simulink model "Architecture_261027_ver9"  (R2026b)
settings: Solver=FixedStepDiscrete  FixedStep=0.005
(part 1 of 2)
settings Model: DataDictionary=Architecture_ver00_dict.sldd  Creator=user  LastModifiedBy=user
settings OptimizationCC: DefaultParameterBehavior=Inlined  DifferentSizesBufferReuse=on  EfficientFloat2IntCast=on  EfficientTunableParamExpr=on  GainParamInheritBuiltInType=on  InlineInvariantSignals=on  LifeSpan=1  NoFixptDivByZeroProtection=on  OptimizeBlockOrder=speed  PassReuseOutputArgsAs=Individual arguments  RemoveInternalMemoryZeroInit=on  RemoveRootLevelIOMemoryZeroInit=on  UseDivisionForNetSlopeComputation=on  UseFloatMulNetSlope=on
settings DebuggingCC: ParameterTunabilityLossMsg=error
settings HardwareCC: ProdHWDeviceType=Infineon->TriCore  ProdLargestAtomicFloat=None  ProdLongLongMode=on
settings SFSimCC: MATLABDynamicMemAlloc=off
settings RTWCC: DataTypeReplacement=CDataTypesFixedWidth  Description=Embedded Coder  GPUComputeCapability=5.0  GenCodeOnly=on  SystemTargetFile=ert.tlc  TemplateMakefile=ert_default_tmf
settings CodeAppCC: ForceParamTrailComments=on  IgnoreCustomStorageClasses=off  InsertBlockDesc=on  OperatorAnnotations=on  SFDataObjDesc=on  SimulinkDataObjDesc=on
settings ERTTargetCC: CombineSignalStateStructs=on  ERTFilePackagingFormat=CompactWithDataFile  IncludeMdlTerminateFcn=off  MaxIdInt16=INT16_MAX  MaxIdInt32=INT32_MAX  MaxIdInt64=INT64_MAX  MaxIdInt8=INT8_MAX  MaxIdUint16=UINT16_MAX  MaxIdUint32=UINT32_MAX  MaxIdUint64=UINT64_MAX  MaxIdUint8=UINT8_MAX  MinIdInt16=INT16_MIN  MinIdInt32=INT32_MIN  MinIdInt64=INT64_MIN  MinIdInt8=INT8_MIN  SupportAbsoluteTime=off  SupportComplex=off  SupportNonFinite=off  SuppressErrorStatus=on

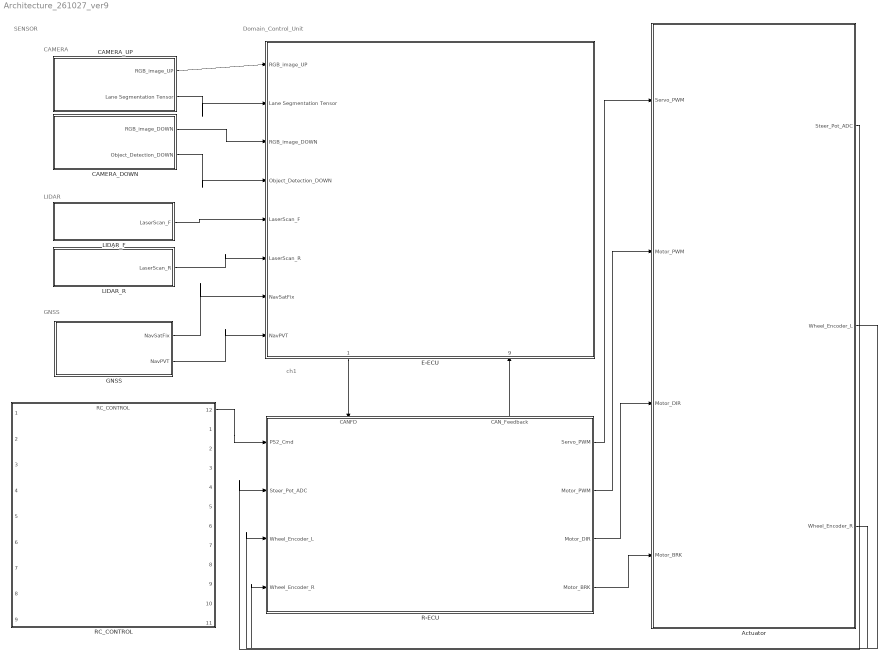
== system Architecture_261027_ver9 ==
  note: ch1
  note: Domain_Control_Unit
  note: SENSOR
  note: CAMERA
  note: GNSS
  note: LIDAR
  Actuator : Subsystem
      settings: PortSchema="{\"entries\":[{\"content\":{\"headerSize\":26,\"margin\":15,\"minimumSpacing\":25,\"sides\":[{\"content\":{\"connectorIds\":[\"In1\",\"In2\",\"In4\",\"In3\"]},\"type\":\"ConnectorPlacement.EquallySpacedRectSide\",\"uuid\":\"5be6b78a-1fb5-4892-a059-20486cb8da03\"},{\"content\":{\"connectorIds\":[\"Out2\",\"Out1\",\"Out3\"],\"side\":\"RIGHT\"},\"type\":\"ConnectorPlacement.EquallySpacedRectSide\",\"uuid\":\"6033bdc5-529e-4fd7-96df-de1a61a0c34f\"},{\"content\":{\"side\":\"TOP\"},\"type\":\"ConnectorPlacement.EquallySpacedRectSide\",\"uuid\":\"4d265f78-1951-4f58-a661-9dd8a9ad83fa\"}]},\"type\":\"ConnectorPlacement.EquallySpacedConnector\",\"uuid\":\"a5be31a5-398c-4cfa-a3f1-90989462f386\"}],\"packageUris\":[\"http://schema.mathworks.com/mf0/Connector/R2020b\"],\"version\":\"1.0\"}"
  CAMERA_DOWN : Subsystem
      settings: PortSchema="{\"entries\":[{\"content\":{\"headerSize\":26,\"margin\":15,\"minimumSpacing\":25,\"sides\":[{\"content\":{},\"type\":\"ConnectorPlacement.EquallySpacedRectSide\",\"uuid\":\"5be6b78a-1fb5-4892-a059-20486cb8da03\"},{\"content\":{\"connectorIds\":[\"Out1\",\"Out2\"],\"side\":\"RIGHT\"},\"type\":\"ConnectorPlacement.EquallySpacedRectSide\",\"uuid\":\"6033bdc5-529e-4fd7-96df-de1a61a0c34f\"},{\"content\":{\"side\":\"TOP\"},\"type\":\"ConnectorPlacement.EquallySpacedRectSide\",\"uuid\":\"4d265f78-1951-4f58-a661-9dd8a9ad83fa\"}]},\"type\":\"ConnectorPlacement.EquallySpacedConnector\",\"uuid\":\"a5be31a5-398c-4cfa-a3f1-90989462f386\"}],\"packageUris\":[\"http://schema.mathworks.com/mf0/Connector/R2020b\"],\"version\":\"1.0\"}"
  CAMERA_UP : Subsystem
      settings: PortSchema="{\"entries\":[{\"content\":{\"headerSize\":26,\"margin\":15,\"minimumSpacing\":25,\"sides\":[{\"content\":{},\"type\":\"ConnectorPlacement.EquallySpacedRectSide\",\"uuid\":\"5be6b78a-1fb5-4892-a059-20486cb8da03\"},{\"content\":{\"connectorIds\":[\"Out1\",\"Out2\"],\"side\":\"RIGHT\"},\"type\":\"ConnectorPlacement.EquallySpacedRectSide\",\"uuid\":\"6033bdc5-529e-4fd7-96df-de1a61a0c34f\"},{\"content\":{\"side\":\"TOP\"},\"type\":\"ConnectorPlacement.EquallySpacedRectSide\",\"uuid\":\"4d265f78-1951-4f58-a661-9dd8a9ad83fa\"}]},\"type\":\"ConnectorPlacement.EquallySpacedConnector\",\"uuid\":\"a5be31a5-398c-4cfa-a3f1-90989462f386\"}],\"packageUris\":[\"http://schema.mathworks.com/mf0/Connector/R2020b\"],\"version\":\"1.0\"}"
  E-ECU : Subsystem
      settings: PortSchema="{\"entries\":[{\"content\":{\"headerSize\":26,\"margin\":15,\"minimumSpacing\":25,\"sides\":[{\"content\":{\"connectorIds\":[\"In1\",\"In2\",\"In3\",\"In4\",\"In5\",\"In6\",\"In7\",\"In8\"]},\"type\":\"ConnectorPlacement.EquallySpacedRectSide\",\"uuid\":\"10eeddd2-005b-4c36-905d-85150b5a76ba\"},{\"content\":{\"side\":\"RIGHT\"},\"type\":\"ConnectorPlacement.EquallySpacedRectSide\",\"uuid\":\"bedc3a09-ff49-49cc-a7fa-ee3f02f55a8a\"},{\"content\":{\"side\":\"TOP\"},\"type\":\"ConnectorPlacement.EquallySpacedRectSide\",\"uuid\":\"08175ed9-a39d-44a1-a51d-de8180bc2cb7\"},{\"content\":{\"connectorIds\":[\"Out1\",\"In9\"],\"side\":\"BOTTOM\"},\"type\":\"ConnectorPlacement.EquallySpacedRectSide\",\"uuid\":\"733d255f-bca5-45f8-986d-3d6c4c00fa39\"}]},\"type\":\"ConnectorPlacement.EquallySpacedConnector\",\"uuid\":\"c3651b75-d651-4d18-be21-a5b7754dce1a\"}],\"packageUris\":[\"http://schema.mathworks.com/mf0/Connector/R2020b\"],\"version\":\"1.0\"}"
  GNSS : Subsystem
      settings: PortSchema="{\"entries\":[{\"content\":{\"headerSize\":26,\"margin\":15,\"minimumSpacing\":25,\"sides\":[{\"content\":{},\"type\":\"ConnectorPlacement.EquallySpacedRectSide\",\"uuid\":\"5be6b78a-1fb5-4892-a059-20486cb8da03\"},{\"content\":{\"connectorIds\":[\"Out1\",\"Out2\"],\"side\":\"RIGHT\"},\"type\":\"ConnectorPlacement.EquallySpacedRectSide\",\"uuid\":\"6033bdc5-529e-4fd7-96df-de1a61a0c34f\"},{\"content\":{\"side\":\"TOP\"},\"type\":\"ConnectorPlacement.EquallySpacedRectSide\",\"uuid\":\"4d265f78-1951-4f58-a661-9dd8a9ad83fa\"}]},\"type\":\"ConnectorPlacement.EquallySpacedConnector\",\"uuid\":\"a5be31a5-398c-4cfa-a3f1-90989462f386\"}],\"packageUris\":[\"http://schema.mathworks.com/mf0/Connector/R2020b\"],\"version\":\"1.0\"}"
  LIDAR_F : Subsystem
      settings: PortSchema="{\"entries\":[{\"content\":{\"headerSize\":26,\"margin\":15,\"minimumSpacing\":25,\"sides\":[{\"content\":{},\"type\":\"ConnectorPlacement.EquallySpacedRectSide\",\"uuid\":\"5be6b78a-1fb5-4892-a059-20486cb8da03\"},{\"content\":{\"connectorIds\":[\"Out1\"],\"side\":\"RIGHT\"},\"type\":\"ConnectorPlacement.EquallySpacedRectSide\",\"uuid\":\"6033bdc5-529e-4fd7-96df-de1a61a0c34f\"},{\"content\":{\"side\":\"TOP\"},\"type\":\"ConnectorPlacement.EquallySpacedRectSide\",\"uuid\":\"4d265f78-1951-4f58-a661-9dd8a9ad83fa\"}]},\"type\":\"ConnectorPlacement.EquallySpacedConnector\",\"uuid\":\"a5be31a5-398c-4cfa-a3f1-90989462f386\"}],\"packageUris\":[\"http://schema.mathworks.com/mf0/Connector/R2020b\"],\"version\":\"1.0\"}"
  LIDAR_R : Subsystem
      settings: PortSchema="{\"entries\":[{\"content\":{\"headerSize\":26,\"margin\":15,\"minimumSpacing\":25,\"sides\":[{\"content\":{},\"type\":\"ConnectorPlacement.EquallySpacedRectSide\",\"uuid\":\"5be6b78a-1fb5-4892-a059-20486cb8da03\"},{\"content\":{\"connectorIds\":[\"Out1\"],\"side\":\"RIGHT\"},\"type\":\"ConnectorPlacement.EquallySpacedRectSide\",\"uuid\":\"6033bdc5-529e-4fd7-96df-de1a61a0c34f\"},{\"content\":{\"side\":\"TOP\"},\"type\":\"ConnectorPlacement.EquallySpacedRectSide\",\"uuid\":\"4d265f78-1951-4f58-a661-9dd8a9ad83fa\"}]},\"type\":\"ConnectorPlacement.EquallySpacedConnector\",\"uuid\":\"a5be31a5-398c-4cfa-a3f1-90989462f386\"}],\"packageUris\":[\"http://schema.mathworks.com/mf0/Connector/R2020b\"],\"version\":\"1.0\"}"
  R-ECU : Subsystem
      settings: PortSchema="{\"entries\":[{\"content\":{\"headerSize\":26,\"margin\":15,\"minimumSpacing\":25,\"sides\":[{\"content\":{\"connectorIds\":[\"In1\",\"In3\",\"In2\",\"In4\"]},\"type\":\"ConnectorPlacement.EquallySpacedRectSide\",\"uuid\":\"5be6b78a-1fb5-4892-a059-20486cb8da03\"},{\"content\":{\"connectorIds\":[\"Out2\",\"Out4\",\"Out3\",\"Out5\"],\"side\":\"RIGHT\"},\"type\":\"ConnectorPlacement.EquallySpacedRectSide\",\"uuid\":\"6033bdc5-529e-4fd7-96df-de1a61a0c34f\"},{\"content\":{\"connectorIds\":[\"In5\",\"Out1\"],\"side\":\"TOP\"},\"type\":\"ConnectorPlacement.EquallySpacedRectSide\",\"uuid\":\"4d265f78-1951-4f58-a661-9dd8a9ad83fa\"}]},\"type\":\"ConnectorPlacement.EquallySpacedConnector\",\"uuid\":\"a5be31a5-398c-4cfa-a3f1-90989462f386\"}],\"packageUris\":[\"http://schema.mathworks.com/mf0/Connector/R2020b\"],\"version\":\"1.0\"}"
  RC_CONTROL : ModelReference  ModelNameDialog=RC_CONTROL  SimulationMode=Normal  ModelReferenceVersion=1.10
      settings: PortSchema="{\"entries\":[{\"content\":{\"headerSize\":38,\"margin\":15,\"minimumSpacing\":25,\"sides\":[{\"content\":{\"connectorIds\":[\"In1\",\"In2\",\"In3\",\"In4\",\"In5\",\"In6\",\"In7\",\"In8\",\"In9\"]},\"type\":\"ConnectorPlacement.EquallySpacedRectSide\",\"uuid\":\"f8644c43-7de7-4551-975f-61d7214ac11a\"},{\"content\":{\"connectorIds\":[\"Out12\",\"Out1\",\"Out2\",\"Out3\",\"Out4\",\"Out5\",\"Out6\",\"Out7\",\"Out8\",\"Out9\",\"Out10\",\"Out11\"],\"side\":\"RIGHT\"},\"type\":\"ConnectorPlacement.EquallySpacedRectSide\",\"uuid\":\"f00a2047-0f06-437d-84ca-9ac4a3f2c44a\"},{\"content\":{\"side\":\"TOP\"},\"type\":\"ConnectorPlacement.EquallySpacedRectSide\",\"uuid\":\"162e5f72-53e9-4ab8-ad74-bc845fd36bb8\"}]},\"type\":\"ConnectorPlacement.EquallySpacedConnector\",\"uuid\":\"4927cb8c-a923-4407-aae2-156d09df746b\"}],\"packageUris\":[\"http://schema.mathworks.com/mf0/Connector/R2020b\"],\"version\":\"1.0\"}"
  wires:
  R-ECU/2(Servo_PWM) -> Actuator/1(Servo_PWM)
  R-ECU/4(Motor_PWM) -> Actuator/2(Motor_PWM)
  R-ECU/5(Motor_BRK) -> Actuator/3(Motor_BRK)
  Actuator/1(Wheel_Encoder_L) -> R-ECU/2(Wheel_Encoder_L)
  Actuator/2(Steer_Pot_ADC) -> R-ECU/3(Steer_Pot_ADC)
  R-ECU/1(CAN_Feedback) -> E-ECU/9("  ")
  E-ECU/1("   ") -> R-ECU/5(CANFD)
  Actuator/3(Wheel_Encoder_R) -> R-ECU/4(Wheel_Encoder_R)
  R-ECU/3(Motor_DIR) -> Actuator/4(Motor_DIR)
  LIDAR_F/1(LaserScan_F) -> E-ECU/5(LaserScan_F)
  LIDAR_R/1(LaserScan_R) -> E-ECU/6(LaserScan_R)
  GNSS/1("NavSatFix ") -> E-ECU/7("NavSatFix ")
  GNSS/2(NavPVT) -> E-ECU/8(NavPVT)
  CAMERA_UP/1(RGB_image_UP) -> E-ECU/1(RGB_image_UP)
  CAMERA_DOWN/1(RGB_image_DOWN) -> E-ECU/3(RGB_image_DOWN)
  CAMERA_DOWN/2(Object_Detection_DOWN) -> E-ECU/4(Object_Detection_DOWN)
  CAMERA_UP/2(Lane Segmentation Tensor) -> E-ECU/2(Lane Segmentation Tensor)
  RC_CONTROL/12 -> R-ECU/1(PS2_Cmd)

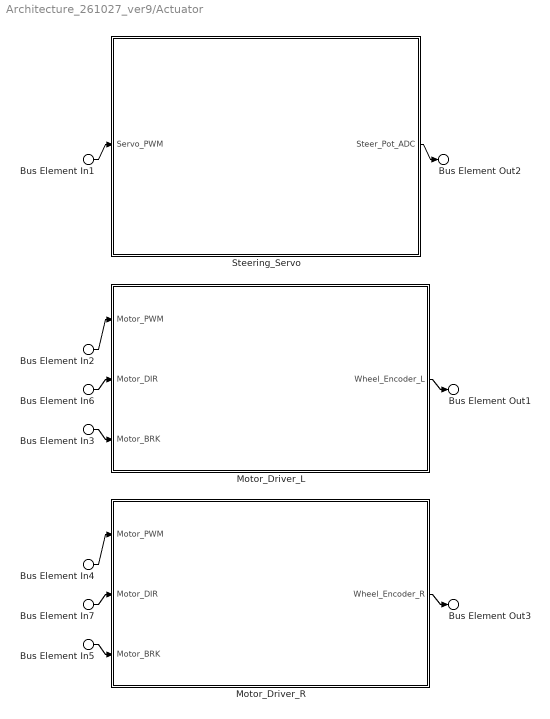
== system Architecture_261027_ver9/Actuator ==
  Bus Element In1 : Inport  PortName=Servo_PWM
  Bus Element In2 : Inport  Port=2  PortName=Motor_PWM
  Bus Element In4 : Inport  Port=2  PortName=Motor_PWM
  Bus Element In3 : Inport  Port=3  PortName=Motor_BRK
  Bus Element In5 : Inport  Port=3  PortName=Motor_BRK
  Bus Element In6 : Inport  Port=4  PortName=Motor_DIR
  Bus Element In7 : Inport  Port=4  PortName=Motor_DIR
  Motor_Driver_L : Subsystem
      settings: PortSchema="{\"entries\":[{\"content\":{\"headerSize\":26,\"margin\":15,\"minimumSpacing\":25,\"sides\":[{\"content\":{\"connectorIds\":[\"In1\",\"In2\",\"In3\"]},\"type\":\"ConnectorPlacement.EquallySpacedRectSide\",\"uuid\":\"5be6b78a-1fb5-4892-a059-20486cb8da03\"},{\"content\":{\"connectorIds\":[\"Out1\"],\"side\":\"RIGHT\"},\"type\":\"ConnectorPlacement.EquallySpacedRectSide\",\"uuid\":\"6033bdc5-529e-4fd7-96df-de1a61a0c34f\"},{\"content\":{\"side\":\"TOP\"},\"type\":\"ConnectorPlacement.EquallySpacedRectSide\",\"uuid\":\"4d265f78-1951-4f58-a661-9dd8a9ad83fa\"}]},\"type\":\"ConnectorPlacement.EquallySpacedConnector\",\"uuid\":\"a5be31a5-398c-4cfa-a3f1-90989462f386\"}],\"packageUris\":[\"http://schema.mathworks.com/mf0/Connector/R2020b\"],\"version\":\"1.0\"}"
  Motor_Driver_R : Subsystem
      settings: PortSchema="{\"entries\":[{\"content\":{\"headerSize\":26,\"margin\":15,\"minimumSpacing\":25,\"sides\":[{\"content\":{\"connectorIds\":[\"In1\",\"In2\",\"In3\"]},\"type\":\"ConnectorPlacement.EquallySpacedRectSide\",\"uuid\":\"5be6b78a-1fb5-4892-a059-20486cb8da03\"},{\"content\":{\"connectorIds\":[\"Out1\"],\"side\":\"RIGHT\"},\"type\":\"ConnectorPlacement.EquallySpacedRectSide\",\"uuid\":\"6033bdc5-529e-4fd7-96df-de1a61a0c34f\"},{\"content\":{\"side\":\"TOP\"},\"type\":\"ConnectorPlacement.EquallySpacedRectSide\",\"uuid\":\"4d265f78-1951-4f58-a661-9dd8a9ad83fa\"}]},\"type\":\"ConnectorPlacement.EquallySpacedConnector\",\"uuid\":\"a5be31a5-398c-4cfa-a3f1-90989462f386\"}],\"packageUris\":[\"http://schema.mathworks.com/mf0/Connector/R2020b\"],\"version\":\"1.0\"}"
  Steering_Servo : Subsystem
      settings: PortSchema="{\"entries\":[{\"content\":{\"headerSize\":26,\"margin\":15,\"minimumSpacing\":25,\"sides\":[{\"content\":{\"connectorIds\":[\"In1\"]},\"type\":\"ConnectorPlacement.EquallySpacedRectSide\",\"uuid\":\"5be6b78a-1fb5-4892-a059-20486cb8da03\"},{\"content\":{\"connectorIds\":[\"Out1\"],\"side\":\"RIGHT\"},\"type\":\"ConnectorPlacement.EquallySpacedRectSide\",\"uuid\":\"6033bdc5-529e-4fd7-96df-de1a61a0c34f\"},{\"content\":{\"side\":\"TOP\"},\"type\":\"ConnectorPlacement.EquallySpacedRectSide\",\"uuid\":\"4d265f78-1951-4f58-a661-9dd8a9ad83fa\"}]},\"type\":\"ConnectorPlacement.EquallySpacedConnector\",\"uuid\":\"a5be31a5-398c-4cfa-a3f1-90989462f386\"}],\"packageUris\":[\"http://schema.mathworks.com/mf0/Connector/R2020b\"],\"version\":\"1.0\"}"
  Bus Element Out1 : Outport  PortName=Wheel_Encoder_L
  Bus Element Out2 : Outport  Port=2  PortName=Steer_Pot_ADC
  Bus Element Out3 : Outport  Port=3  PortName=Wheel_Encoder_R
  wires:
  Motor_Driver_L/1(Wheel_Encoder_L) -> Bus Element Out1/1
  Bus Element In1/1 -> Steering_Servo/1(Servo_PWM)
  Bus Element In2/1 -> Motor_Driver_L/1(Motor_PWM)
  Bus Element In3/1 -> Motor_Driver_L/3(Motor_BRK)
  Steering_Servo/1(Steer_Pot_ADC) -> Bus Element Out2/1
  Motor_Driver_R/1(Wheel_Encoder_R) -> Bus Element Out3/1
  Bus Element In4/1 -> Motor_Driver_R/1(Motor_PWM)
  Bus Element In5/1 -> Motor_Driver_R/3(Motor_BRK)
  Bus Element In6/1 -> Motor_Driver_L/2(Motor_DIR)
  Bus Element In7/1 -> Motor_Driver_R/2(Motor_DIR)

== system Architecture_261027_ver9/CAMERA_DOWN ==
  Bus Element Out1 : Outport  PortName=RGB_image_DOWN
  Bus Element Out2 : Outport  Port=2  PortName=Object_Detection_DOWN

== system Architecture_261027_ver9/CAMERA_UP ==
  Bus Element Out1 : Outport  PortName=RGB_image_UP
  Bus Element Out2 : Outport  Port=2  PortName=Lane Segmentation Tensor

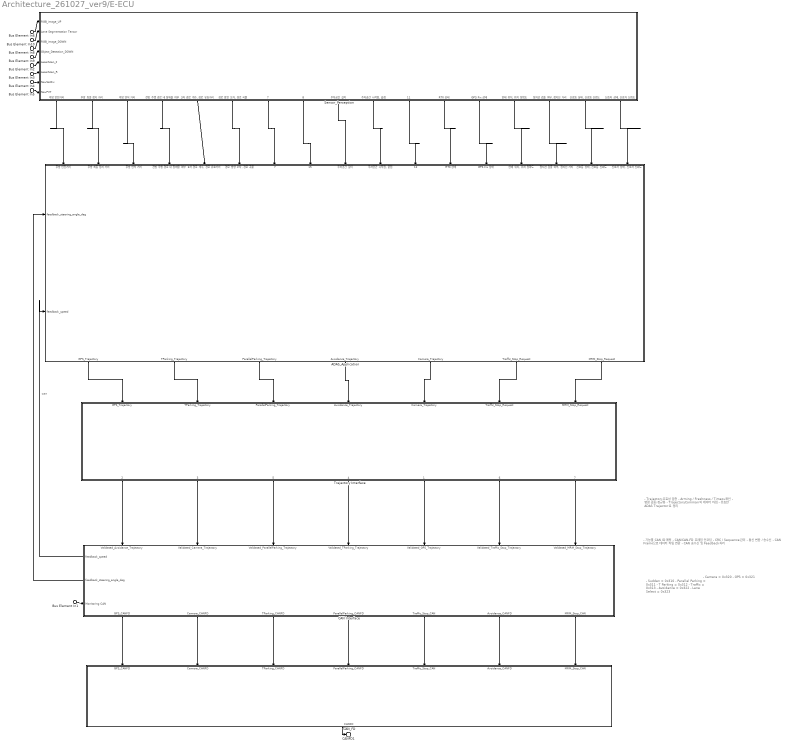
== system Architecture_261027_ver9/E-ECU ==
  note: can
  note: - 기능별 CAN ID 매핑
      | - CAN/CAN-FD 프레임 인코딩
      | - CRC / Sequence 관리
      | - 통신 변환 / 송수신
      | - CAN Frame으로 데이터 타입 변환
      | - CAN 송수신 및 Feedback 처리
  note: - Trajectory 유효성 검증
      | - Arming / Freshness / Timeout 확인
      | - 명령 검증/정규화
      | - TrajectoryCommand의 데이터 타입
      | - 유효한 ADAS Trajectory로 정리
  note: - Camera = 0x320
      | - GPS = 0x321
  note: - Sudden = 0x310
      | - Parallel Parking = 0x311
      | - T Parking = 0x312
      | - Traffic = 0x313
      | - Avoidance = 0x322
      | - Lane Select = 0x323
  Bus Element In6 : Inport  PortName=RGB_image_UP
  Bus Element In10 : Inport  Port=2  PortName=Lane Segmentation Tensor
  Bus Element In8 : Inport  Port=3  PortName=RGB_image_DOWN
  Bus Element In9 : Inport  Port=4  PortName=Object_Detection_DOWN
  Bus Element In2 : Inport  Port=5  PortName=LaserScan_F
  Bus Element In3 : Inport  Port=6  PortName=LaserScan_R
  Bus Element In4 : Inport  Port=7  PortName=NavSatFix
  Bus Element In5 : Inport  Port=8  PortName=NavPVT
  Bus Element In1 : Inport  Port=9  PortName=""
  ADAS_Application : Subsystem
      settings: PortSchema="{\"entries\":[{\"content\":{\"headerSize\":26,\"margin\":15,\"minimumSpacing\":25,\"sides\":[{\"content\":{\"connectorIds\":[\"In5\",\"In8\"]},\"type\":\"ConnectorPlacement.EquallySpacedRectSide\",\"uuid\":\"47be2e05-6379-4865-963e-e2af5bd447f4\"},{\"content\":{\"side\":\"RIGHT\"},\"type\":\"ConnectorPlacement.EquallySpacedRectSide\",\"uuid\":\"eee9a279-489d-42b1-868c-6501adb5baa4\"},{\"content\":{\"connectorIds\":[\"In19\",\"In18\",\"In17\",\"In16\",\"In4\",\"In6\",\"In7\",\"In15\",\"In14\",\"In13\",\"In12\",\"In11\",\"In10\",\"In9\",\"In2\",\"In1\",\"In3\"],\"side\":\"TOP\"},\"type\":\"ConnectorPlacement.EquallySpacedRectSide\",\"uuid\":\"1fb23197-7de0-4afe-988c-73e75d3e5644\"},{\"content\":{\"connectorIds\":[\"Out1\",\"Out2\",\"Out3\",\"Out4\",\"Out5\",\"Out7\",\"Out6\"],\"side\":\"BOTTOM\"},\"type\":\"ConnectorPlacement.EquallySpacedRectSide\",\"uuid\":\"4316405c-13a5-45fc-a271-26a0825c33e2\"}]},\"type\":\"ConnectorPlacement.EquallySpacedConnector\",\"uuid\":\"0ef4e16f-7381-4a8b-98d2-b00a0700ad12\"}],\"packageUris\":[\"http://schema.mathworks.com/mf0/Connector/R2020b\"],\"version\":\"1.0\"}"
  CAN Interface : Subsystem
      settings: PortSchema="{\"entries\":[{\"content\":{\"headerSize\":26,\"margin\":15,\"minimumSpacing\":25,\"sides\":[{\"content\":{\"connectorIds\":[\"Out1\",\"Out2\",\"In1\"]},\"type\":\"ConnectorPlacement.EquallySpacedRectSide\",\"uuid\":\"47be2e05-6379-4865-963e-e2af5bd447f4\"},{\"content\":{\"side\":\"RIGHT\"},\"type\":\"ConnectorPlacement.EquallySpacedRectSide\",\"uuid\":\"eee9a279-489d-42b1-868c-6501adb5baa4\"},{\"content\":{\"connectorIds\":[\"In8\",\"In3\",\"In5\",\"In4\",\"In2\",\"In6\",\"In7\"],\"side\":\"TOP\"},\"type\":\"ConnectorPlacement.EquallySpacedRectSide\",\"uuid\":\"1fb23197-7de0-4afe-988c-73e75d3e5644\"},{\"content\":{\"connectorIds\":[\"Out3\",\"Out4\",\"Out5\",\"Out6\",\"Out8\",\"Out7\",\"Out9\"],\"side\":\"BOTTOM\"},\"type\":\"ConnectorPlacement.EquallySpacedRectSide\",\"uuid\":\"b394a130-1425-4269-a0f2-9cc8deadb9ec\"}]},\"type\":\"ConnectorPlacement.EquallySpacedConnector\",\"uuid\":\"0ef4e16f-7381-4a8b-98d2-b00a0700ad12\"}],\"packageUris\":[\"http://schema.mathworks.com/mf0/Connector/R2020b\"],\"version\":\"1.0\"}"
  CAN_FD : Subsystem
      settings: PortSchema="{\"entries\":[{\"content\":{\"headerSize\":26,\"margin\":15,\"minimumSpacing\":25,\"sides\":[{\"content\":{},\"type\":\"ConnectorPlacement.EquallySpacedRectSide\",\"uuid\":\"47be2e05-6379-4865-963e-e2af5bd447f4\"},{\"content\":{\"side\":\"RIGHT\"},\"type\":\"ConnectorPlacement.EquallySpacedRectSide\",\"uuid\":\"eee9a279-489d-42b1-868c-6501adb5baa4\"},{\"content\":{\"connectorIds\":[\"In3\",\"In4\",\"In5\",\"In6\",\"In2\",\"In7\",\"In1\"],\"side\":\"TOP\"},\"type\":\"ConnectorPlacement.EquallySpacedRectSide\",\"uuid\":\"1fb23197-7de0-4afe-988c-73e75d3e5644\"},{\"content\":{\"connectorIds\":[\"Out1\"],\"side\":\"BOTTOM\"},\"type\":\"ConnectorPlacement.EquallySpacedRectSide\",\"uuid\":\"43bc4a7e-8fe5-43f2-b7c3-d50d46211fbc\"}]},\"type\":\"ConnectorPlacement.EquallySpacedConnector\",\"uuid\":\"0ef4e16f-7381-4a8b-98d2-b00a0700ad12\"}],\"packageUris\":[\"http://schema.mathworks.com/mf0/Connector/R2020b\"],\"version\":\"1.0\"}"
  Sensor_Perception : Subsystem
      settings: PortSchema="{\"entries\":[{\"content\":{\"headerSize\":26,\"margin\":15,\"minimumSpacing\":25,\"sides\":[{\"content\":{\"connectorIds\":[\"In1\",\"In2\",\"In3\",\"In4\",\"In5\",\"In6\",\"In8\",\"In7\"]},\"type\":\"ConnectorPlacement.EquallySpacedRectSide\",\"uuid\":\"833e2261-d969-4b6b-a2a0-d6d2d41b6c97\"},{\"content\":{\"side\":\"RIGHT\"},\"type\":\"ConnectorPlacement.EquallySpacedRectSide\",\"uuid\":\"a75417d5-389f-432a-8681-855d3d99c66c\"},{\"content\":{\"side\":\"TOP\"},\"type\":\"ConnectorPlacement.EquallySpacedRectSide\",\"uuid\":\"4b4e12bc-525c-4fca-adf7-0dacf20b4e90\"},{\"content\":{\"connectorIds\":[\"Out1\",\"Out2\",\"Out3\",\"Out4\",\"Out5\",\"Out6\",\"Out7\",\"Out8\",\"Out9\",\"Out10\",\"Out11\",\"Out12\",\"Out13\",\"Out15\",\"Out16\",\"Out17\",\"Out14\"],\"side\":\"BOTTOM\"},\"type\":\"ConnectorPlacement.EquallySpacedRectSide\",\"uuid\":\"8c2e8235-c7de-4058-b006-d48e7e6bf32d\"}]},\"type\":\"ConnectorPlacement.EquallySpacedConnector\",\"uuid\":\"d54c61eb-5c90-4dca-8a18-d288ca99e2e1\"}],\"packageUris\":[\"http://schema.mathworks.com/mf0/Connector/R2020b\"],\"version\":\"1.0\"}"
  Trajectory Interface : Subsystem
      settings: PortSchema="{\"entries\":[{\"content\":{\"headerSize\":26,\"margin\":15,\"minimumSpacing\":25,\"sides\":[{\"content\":{},\"type\":\"ConnectorPlacement.EquallySpacedRectSide\",\"uuid\":\"47be2e05-6379-4865-963e-e2af5bd447f4\"},{\"content\":{\"side\":\"RIGHT\"},\"type\":\"ConnectorPlacement.EquallySpacedRectSide\",\"uuid\":\"eee9a279-489d-42b1-868c-6501adb5baa4\"},{\"content\":{\"connectorIds\":[\"In1\",\"In2\",\"In3\",\"In4\",\"In5\",\"In6\",\"In7\"],\"side\":\"TOP\"},\"type\":\"ConnectorPlacement.EquallySpacedRectSide\",\"uuid\":\"1fb23197-7de0-4afe-988c-73e75d3e5644\"},{\"content\":{\"connectorIds\":[\"Out2\",\"Out3\",\"Out5\",\"Out4\",\"Out1\",\"Out6\",\"Out7\"],\"side\":\"BOTTOM\"},\"type\":\"ConnectorPlacement.EquallySpacedRectSide\",\"uuid\":\"0687b936-52e7-4e92-b361-bf32be88b9f9\"}]},\"type\":\"ConnectorPlacement.EquallySpacedConnector\",\"uuid\":\"0ef4e16f-7381-4a8b-98d2-b00a0700ad12\"}],\"packageUris\":[\"http://schema.mathworks.com/mf0/Connector/R2020b\"],\"version\":\"1.0\"}"
  CANFD1 : Outport  PortName=""
  wires:
  ADAS_Application/1(GPS_Trajectory) -> Trajectory Interface/1(GPS_Trajectory)
  ADAS_Application/2(TParking_Trajectory) -> Trajectory Interface/2(TParking_Trajectory)
  ADAS_Application/3(ParallelParking_Trajectory) -> Trajectory Interface/3(ParallelParking_Trajectory)
  ADAS_Application/4(Avoidance_Trajectory) -> Trajectory Interface/4(Avoidance_Trajectory)
  ADAS_Application/5(Camera_Trajectory) -> Trajectory Interface/5(Camera_Trajectory)
  Trajectory Interface/1("     ") -> CAN Interface/2(Validated_GPS_Trajectory)
  Trajectory Interface/3("  ") -> CAN Interface/3(Validated_Camera_Trajectory)
  Trajectory Interface/4("    ") -> CAN Interface/4(Validated_TParking_Trajectory)
  Trajectory Interface/5("   ") -> CAN Interface/5(Validated_ParallelParking_Trajectory)
  Trajectory Interface/2(" ") -> CAN Interface/8(Validated_Avoidance_Trajectory)
  CAN_FD/1(CANFD) -> CANFD1/1
  CAN Interface/3(GPS_CANFD) -> CAN_FD/3(GPS_CANFD)
  CAN Interface/4(Camera_CANFD) -> CAN_FD/4(Camera_CANFD)
  CAN Interface/5(TParking_CANFD) -> CAN_FD/5(TParking_CANFD)
  CAN Interface/6(ParallelParking_CANFD) -> CAN_FD/6(ParallelParking_CANFD)
  CAN Interface/7(Avoidance_CANFD) -> CAN_FD/7(Avoidance_CANFD)
  CAN Interface/8(Traffic_Stop_CAN) -> CAN_FD/2(Traffic_Stop_CAN)
  CAN Interface/9(MRM_Stop_CAN) -> CAN_FD/1(MRM_Stop_CAN)
  CAN Interface/1(feedback_speed) -> ADAS_Application/8(feedback_speed)
  CAN Interface/2(feedback_steering_angle_deg) -> ADAS_Application/5(feedback_steering_angle_deg)
  Bus Element In1/1 -> CAN Interface/1(Monitoring CAN)
  ADAS_Application/7(Traffic_Stop_Request) -> Trajectory Interface/6(Traffic_Stop_Request)
  ADAS_Application/6(MRM_Stop_Request) -> Trajectory Interface/7(MRM_Stop_Request)
  Trajectory Interface/6("      ") -> CAN Interface/6(Validated_Traffic_Stop_Trajectory)
  Trajectory Interface/7("        ") -> CAN Interface/7(Validated_MRM_Stop_Trajectory)
  Sensor_Perception/17("신호등 상태, 신호등 신뢰도") -> ADAS_Application/1("신호등 상태, 신호등 신뢰도")
  Sensor_Perception/14("신호차 상태, 신호차 신뢰도") -> ADAS_Application/3("신호차 상태, 신호차 신뢰도")
  Sensor_Perception/16("정지선 검출 여부, 정지선 거리") -> ADAS_Application/2("정지선 검출 여부, 정지선 거리")
  Sensor_Perception/15("현재 위치, 위치 정확도") -> ADAS_Application/9("현재 위치, 위치 정확도")
  Sensor_Perception/13(GPS Fix 상태) -> ADAS_Application/10(GPS Fix 상태)
  Sensor_Perception/12(RTK 상태) -> ADAS_Application/11(RTK 상태)
  Sensor_Perception/11("전방 연석 검출 여부, 측면 연석 거리") -> ADAS_Application/12("전방 연석 검출 여부, 측면 연석 거리")
  Sensor_Perception/10("주차공간 시작점, 끝점") -> ADAS_Application/13("주차공간 시작점, 끝점")
  Sensor_Perception/9(주차공간 길이) -> ADAS_Application/14(주차공간 길이)
  Sensor_Perception/8("전방 장애물 거리, 폭, 좌우 위치") -> ADAS_Application/15("전방 장애물 거리, 폭, 좌우 위치")
  Sensor_Perception/4(전방 주행 경로 내 장애물 여부) -> ADAS_Application/16(전방 주행 경로 내 장애물 여부)
  Sensor_Perception/3(후방 연석 거리) -> ADAS_Application/17(후방 연석 거리)
  Sensor_Perception/2(후방 최종 정지 거리) -> ADAS_Application/18(후방 최종 정지 거리)
  Sensor_Perception/1(후방 안전거리) -> ADAS_Application/19(후방 안전거리)
  Bus Element In6/1 -> Sensor_Perception/1(RGB_image_UP)
  Bus Element In8/1 -> Sensor_Perception/3(RGB_image_DOWN)
  Bus Element In9/1 -> Sensor_Perception/4(Object_Detection_DOWN)
  Bus Element In2/1 -> Sensor_Perception/5(LaserScan_F)
  Bus Element In3/1 -> Sensor_Perception/6(LaserScan_R)
  Bus Element In4/1 -> Sensor_Perception/8("NavSatFix ")
  Bus Element In5/1 -> Sensor_Perception/7(NavPVT)
  Bus Element In10/1 -> Sensor_Perception/2(Lane Segmentation Tensor)
  Sensor_Perception/5("3차 경로 계수, 경로 유효거리") -> ADAS_Application/4("3차 경로 계수, 경로 유효거리")
  Sensor_Perception/6("경로 방향 오차, 경로 곡률") -> ADAS_Application/6("경로 방향 오차, 경로 곡률")
  Sensor_Perception/7("차선/경로 유효 여부, 신뢰도, 차량 횡방향 오차") -> ADAS_Application/7("차선/경로 유효 여부, 신뢰도, 차량 횡방향 오차")

== system Architecture_261027_ver9/GNSS ==
  Bus Element Out1 : Outport  PortName=NavSatFix
  Bus Element Out2 : Outport  Port=2  PortName=NavPVT

== system Architecture_261027_ver9/LIDAR_F ==
  Bus Element Out1 : Outport  PortName=LaserScan_F

== system Architecture_261027_ver9/LIDAR_R ==
  Bus Element Out1 : Outport  PortName=LaserScan_R

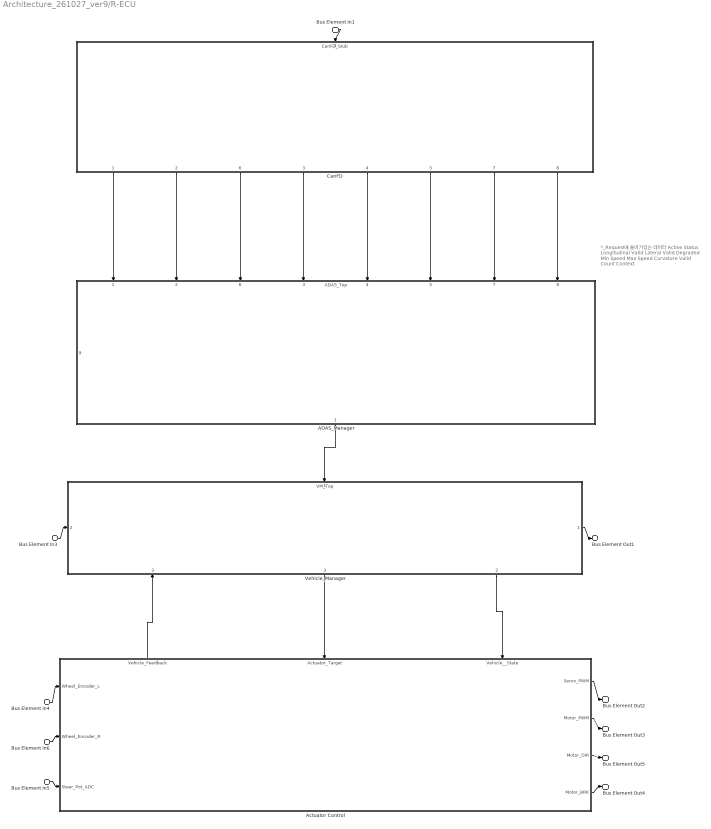
== system Architecture_261027_ver9/R-ECU ==
  note: *_Request에 들어가있는 데이터
      | Active
      | Status
      | Longitudinal Valid
      | Lateral Valid
      | Degraded
      | Min Speed
      | Max Speed
      | Curvature
      | Valid Count
      | Context
  Bus Element In3 : Inport  PortName=PS2_Cmd
  Bus Element In4 : Inport  Port=2  PortName=Wheel_Encoder_L
  Bus Element In5 : Inport  Port=3  PortName=Steer_Pot_ADC
  Bus Element In6 : Inport  Port=4  PortName=Wheel_Encoder_R
  Bus Element In1 : Inport  Port=5  PortName=CANFD
  ADAS_Manager : ModelReference  ModelNameDialog=ADAS_Top  SimulationMode=Normal  ModelReferenceVersion=1.7
      settings: PortSchema="{\"entries\":[{\"content\":{\"headerSize\":38,\"margin\":15,\"minimumSpacing\":25,\"sides\":[{\"content\":{\"connectorIds\":[\"In9\"]},\"type\":\"ConnectorPlacement.EquallySpacedRectSide\",\"uuid\":\"5be6b78a-1fb5-4892-a059-20486cb8da03\"},{\"content\":{\"side\":\"RIGHT\"},\"type\":\"ConnectorPlacement.EquallySpacedRectSide\",\"uuid\":\"6033bdc5-529e-4fd7-96df-de1a61a0c34f\"},{\"content\":{\"connectorIds\":[\"In1\",\"In2\",\"In6\",\"In3\",\"In4\",\"In5\",\"In7\",\"In8\"],\"side\":\"TOP\"},\"type\":\"ConnectorPlacement.EquallySpacedRectSide\",\"uuid\":\"4d265f78-1951-4f58-a661-9dd8a9ad83fa\"},{\"content\":{\"connectorIds\":[\"Out1\"],\"side\":\"BOTTOM\"},\"type\":\"ConnectorPlacement.EquallySpacedRectSide\",\"uuid\":\"98ed4b17-3e59-44a3-acac-4609ccf4a66c\"}]},\"type\":\"ConnectorPlacement.EquallySpacedConnector\",\"uuid\":\"a5be31a5-398c-4cfa-a3f1-90989462f386\"}],\"packageUris\":[\"http://schema.mathworks.com/mf0/Connector/R2020b\"],\"version\":\"1.0\"}"
  Actuator Control : Subsystem
      settings: PortSchema="{\"entries\":[{\"content\":{\"headerSize\":26,\"margin\":15,\"minimumSpacing\":25,\"sides\":[{\"content\":{\"connectorIds\":[\"In3\",\"In4\",\"In5\"]},\"type\":\"ConnectorPlacement.EquallySpacedRectSide\",\"uuid\":\"5be6b78a-1fb5-4892-a059-20486cb8da03\"},{\"content\":{\"connectorIds\":[\"Out3\",\"Out4\",\"Out1\",\"Out5\"],\"side\":\"RIGHT\"},\"type\":\"ConnectorPlacement.EquallySpacedRectSide\",\"uuid\":\"6033bdc5-529e-4fd7-96df-de1a61a0c34f\"},{\"content\":{\"connectorIds\":[\"Out2\",\"In1\",\"In2\"],\"side\":\"TOP\"},\"type\":\"ConnectorPlacement.EquallySpacedRectSide\",\"uuid\":\"4d265f78-1951-4f58-a661-9dd8a9ad83fa\"}]},\"type\":\"ConnectorPlacement.EquallySpacedConnector\",\"uuid\":\"a5be31a5-398c-4cfa-a3f1-90989462f386\"}],\"packageUris\":[\"http://schema.mathworks.com/mf0/Connector/R2020b\"],\"version\":\"1.0\"}"
  CanFD : ModelReference  ModelNameDialog=CanFD_Stub  SimulationMode=Normal  ModelReferenceVersion=1.8
      settings: PortSchema="{\"entries\":[{\"content\":{\"headerSize\":38,\"margin\":15,\"minimumSpacing\":25,\"sides\":[{\"content\":{},\"type\":\"ConnectorPlacement.EquallySpacedRectSide\",\"uuid\":\"6b53cd95-661c-4981-8d03-a3f2c36ff719\"},{\"content\":{\"side\":\"RIGHT\"},\"type\":\"ConnectorPlacement.EquallySpacedRectSide\",\"uuid\":\"a4afb36b-f44c-4b80-af48-0fae29574c12\"},{\"content\":{\"connectorIds\":[\"In1\"],\"side\":\"TOP\"},\"type\":\"ConnectorPlacement.EquallySpacedRectSide\",\"uuid\":\"33efa4fa-6270-4460-be8a-5531e16e9ea1\"},{\"content\":{\"connectorIds\":[\"Out1\",\"Out2\",\"Out6\",\"Out3\",\"Out4\",\"Out5\",\"Out7\",\"Out8\"],\"side\":\"BOTTOM\"},\"type\":\"ConnectorPlacement.EquallySpacedRectSide\",\"uuid\":\"c7bc5dd5-c3ae-484c-bdd0-9cfccd696761\"}]},\"type\":\"ConnectorPlacement.EquallySpacedConnector\",\"uuid\":\"95b4a40c-51bc-41f7-83dc-47ea7edd823b\"}],\"packageUris\":[\"http://schema.mathworks.com/mf0/Connector/R2020b\"],\"version\":\"1.0\"}"
  Vehicle_Manager : ModelReference  ModelNameDialog=VM_Top  SimulationMode=Normal  ModelReferenceVersion=1.13
      settings: PortSchema="{\"entries\":[{\"content\":{\"headerSize\":38,\"margin\":15,\"minimumSpacing\":25,\"sides\":[{\"content\":{\"connectorIds\":[\"In2\"]},\"type\":\"ConnectorPlacement.EquallySpacedRectSide\",\"uuid\":\"5be6b78a-1fb5-4892-a059-20486cb8da03\"},{\"content\":{\"connectorIds\":[\"Out1\"],\"side\":\"RIGHT\"},\"type\":\"ConnectorPlacement.EquallySpacedRectSide\",\"uuid\":\"6033bdc5-529e-4fd7-96df-de1a61a0c34f\"},{\"content\":{\"connectorIds\":[\"In1\"],\"side\":\"TOP\"},\"type\":\"ConnectorPlacement.EquallySpacedRectSide\",\"uuid\":\"4d265f78-1951-4f58-a661-9dd8a9ad83fa\"},{\"content\":{\"connectorIds\":[\"In3\",\"Out3\",\"Out2\"],\"side\":\"BOTTOM\"},\"type\":\"ConnectorPlacement.EquallySpacedRectSide\",\"uuid\":\"080e26dc-87d2-4d1d-9dc9-3d67ba482a61\"}]},\"type\":\"ConnectorPlacement.EquallySpacedConnector\",\"uuid\":\"a5be31a5-398c-4cfa-a3f1-90989462f386\"}],\"packageUris\":[\"http://schema.mathworks.com/mf0/Connector/R2020b\"],\"version\":\"1.0\"}"
  Bus Element Out1 : Outport  PortName=CAN_Feedback
  Bus Element Out2 : Outport  Port=2  PortName=Servo_PWM
  Bus Element Out5 : Outport  Port=3  PortName=Motor_DIR
  Bus Element Out3 : Outport  Port=4  PortName=Motor_PWM
  Bus Element Out4 : Outport  Port=5  PortName=Motor_BRK
  wires:
  Actuator Control/5(Motor_BRK) -> Bus Element Out4/1
  Actuator Control/4(Motor_PWM) -> Bus Element Out3/1
  Actuator Control/3(Servo_PWM) -> Bus Element Out2/1
  Bus Element In4/1 -> Actuator Control/3(Wheel_Encoder_L)
  Bus Element In5/1 -> Actuator Control/5(Steer_Pot_ADC)
  Bus Element In6/1 -> Actuator Control/4(Wheel_Encoder_R)
  Actuator Control/1(Motor_DIR) -> Bus Element Out5/1
  Vehicle_Manager/2 -> Actuator Control/2(Vehicle__State)
  Bus Element In3/1 -> Vehicle_Manager/2
  Actuator Control/2(Vehicle_Feedback) -> Vehicle_Manager/3
  Vehicle_Manager/3 -> Actuator Control/1(Actuator_Target)
  Vehicle_Manager/1 -> Bus Element Out1/1
  ADAS_Manager/1 -> Vehicle_Manager/1
  Bus Element In1/1 -> CanFD/1
  CanFD/3 -> ADAS_Manager/3
  CanFD/1 -> ADAS_Manager/1
  CanFD/6 -> ADAS_Manager/6
  CanFD/2 -> ADAS_Manager/2
  CanFD/7 -> ADAS_Manager/7
  CanFD/5 -> ADAS_Manager/5
  CanFD/4 -> ADAS_Manager/4
  CanFD/8 -> ADAS_Manager/8

== system Architecture_261027_ver9/Actuator/Motor_Driver_L ==
  Bus Element In1 : Inport  PortName=Motor_PWM
  Bus Element In3 : Inport  Port=2  PortName=Motor_DIR
  Bus Element In2 : Inport  Port=3  PortName=Motor_BRK
  Bus Element Out1 : Outport  PortName=Wheel_Encoder_L

== system Architecture_261027_ver9/Actuator/Motor_Driver_R ==
  Bus Element In1 : Inport  PortName=Motor_PWM
  Bus Element In3 : Inport  Port=2  PortName=Motor_DIR
  Bus Element In2 : Inport  Port=3  PortName=Motor_BRK
  Bus Element Out1 : Outport  PortName=Wheel_Encoder_R

== system Architecture_261027_ver9/Actuator/Steering_Servo ==
  Bus Element In1 : Inport  PortName=Servo_PWM
  Bus Element Out1 : Outport  PortName=Steer_Pot_ADC

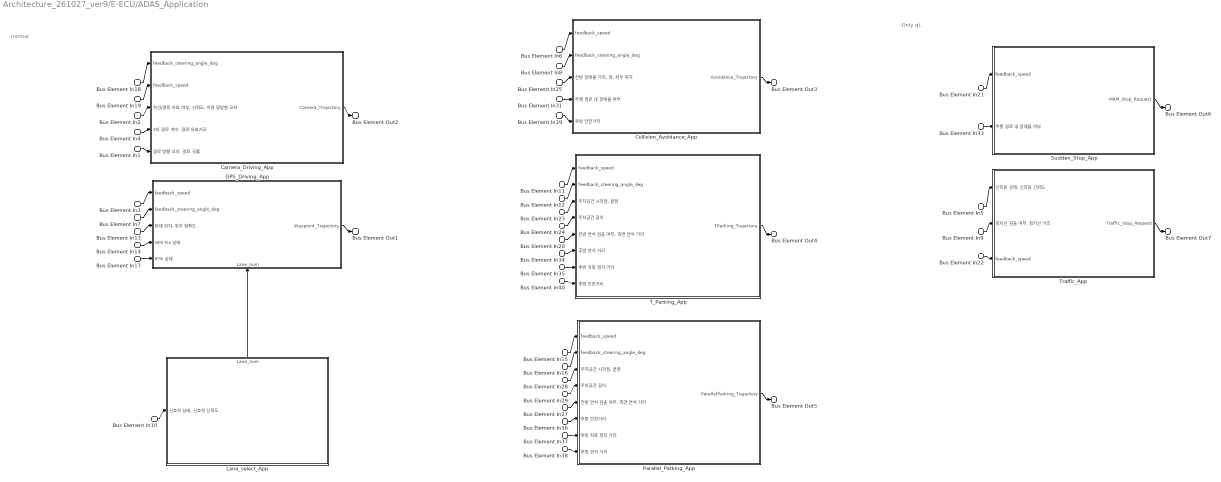
== system Architecture_261027_ver9/E-ECU/ADAS_Application ==
  note: Only qL
  note: normal
  Bus Element In5 : Inport  PortName=신호등 상태, 신호등 신뢰도
  Bus Element In9 : Inport  Port=2  PortName=정지선 검출 여부, 정지선 거리
  Bus Element In10 : Inport  Port=3  PortName=신호차 상태, 신호차 신뢰도
  Bus Element In4 : Inport  Port=4  PortName=3차 경로 계수, 경로 유효거리
  Bus Element In{7..8,12,16,18} (5 alike) : Inport  Port=5  PortName=feedback_steering_angle_deg
  Bus Element In1 : Inport  Port=6  PortName=경로 방향 오차, 경로 곡률
  Bus Element In2 : Inport  Port=7  PortName=차선/경로 유효 여부, 신뢰도, 차량 횡방향 오차
  Bus Element In{3,6,11,15,19,21..22} (7 alike) : Inport  Port=8  PortName=feedback_speed
  Bus Element In13 : Inport  Port=9  PortName=현재 위치, 위치 정확도
  Bus Element In14 : Inport  Port=10  PortName=GPS Fix 상태
  Bus Element In17 : Inport  Port=11  PortName=RTK 상태
  Bus Element In20 : Inport  Port=12  PortName=전방 연석 검출 여부, 측면 연석 거리
  Bus Element In27 : Inport  Port=12  PortName=전방 연석 검출 여부, 측면 연석 거리
  Bus Element In23 : Inport  Port=13  PortName=주차공간 시작점, 끝점
  Bus Element In28 : Inport  Port=13  PortName=주차공간 시작점, 끝점
  Bus Element In24 : Inport  Port=14  PortName=주차공간 길이
  Bus Element In29 : Inport  Port=14  PortName=주차공간 길이
  Bus Element In25 : Inport  Port=15  PortName=전방 장애물 거리, 폭, 좌우 위치
  Bus Element In31 : Inport  Port=16  PortName=전방 주행 경로 내 장애물 여부
  Bus Element In33 : Inport  Port=16  PortName=전방 주행 경로 내 장애물 여부
  Bus Element In34 : Inport  Port=17  PortName=후방 연석 거리
  Bus Element In38 : Inport  Port=17  PortName=후방 연석 거리
  Bus Element In35 : Inport  Port=18  PortName=후방 최종 정지 거리
  Bus Element In37 : Inport  Port=18  PortName=후방 최종 정지 거리
  Bus Element In36 : Inport  Port=19  PortName=후방 안전거리
  Bus Element In39 : Inport  Port=19  PortName=후방 안전거리
  Bus Element In40 : Inport  Port=19  PortName=후방 안전거리
  Camera_Driving_App : Subsystem
      settings: PortSchema="{\"entries\":[{\"content\":{\"headerSize\":26,\"margin\":15,\"minimumSpacing\":25,\"sides\":[{\"content\":{\"connectorIds\":[\"In1\",\"In2\",\"In3\",\"In4\",\"In5\"]},\"type\":\"ConnectorPlacement.EquallySpacedRectSide\",\"uuid\":\"47be2e05-6379-4865-963e-e2af5bd447f4\"},{\"content\":{\"connectorIds\":[\"Out1\"],\"side\":\"RIGHT\"},\"type\":\"ConnectorPlacement.EquallySpacedRectSide\",\"uuid\":\"eee9a279-489d-42b1-868c-6501adb5baa4\"},{\"content\":{\"side\":\"TOP\"},\"type\":\"ConnectorPlacement.EquallySpacedRectSide\",\"uuid\":\"1fb23197-7de0-4afe-988c-73e75d3e5644\"}]},\"type\":\"ConnectorPlacement.EquallySpacedConnector\",\"uuid\":\"0ef4e16f-7381-4a8b-98d2-b00a0700ad12\"}],\"packageUris\":[\"http://schema.mathworks.com/mf0/Connector/R2020b\"],\"version\":\"1.0\"}"
  Collision_Avoidance_App : Subsystem
      settings: PortSchema="{\"entries\":[{\"content\":{\"headerSize\":26,\"margin\":15,\"minimumSpacing\":25,\"sides\":[{\"content\":{\"connectorIds\":[\"In1\",\"In2\",\"In3\",\"In4\",\"In5\"]},\"type\":\"ConnectorPlacement.EquallySpacedRectSide\",\"uuid\":\"47be2e05-6379-4865-963e-e2af5bd447f4\"},{\"content\":{\"connectorIds\":[\"Out1\"],\"side\":\"RIGHT\"},\"type\":\"ConnectorPlacement.EquallySpacedRectSide\",\"uuid\":\"eee9a279-489d-42b1-868c-6501adb5baa4\"},{\"content\":{\"side\":\"TOP\"},\"type\":\"ConnectorPlacement.EquallySpacedRectSide\",\"uuid\":\"1fb23197-7de0-4afe-988c-73e75d3e5644\"}]},\"type\":\"ConnectorPlacement.EquallySpacedConnector\",\"uuid\":\"0ef4e16f-7381-4a8b-98d2-b00a0700ad12\"}],\"packageUris\":[\"http://schema.mathworks.com/mf0/Connector/R2020b\"],\"version\":\"1.0\"}"
  GPS_Driving_App : Subsystem
      settings: PortSchema="{\"entries\":[{\"content\":{\"headerSize\":26,\"margin\":15,\"minimumSpacing\":25,\"sides\":[{\"content\":{\"connectorIds\":[\"In2\",\"In6\",\"In3\",\"In4\",\"In5\"]},\"type\":\"ConnectorPlacement.EquallySpacedRectSide\",\"uuid\":\"47be2e05-6379-4865-963e-e2af5bd447f4\"},{\"content\":{\"connectorIds\":[\"Out1\"],\"side\":\"RIGHT\"},\"type\":\"ConnectorPlacement.EquallySpacedRectSide\",\"uuid\":\"eee9a279-489d-42b1-868c-6501adb5baa4\"},{\"content\":{\"side\":\"TOP\"},\"type\":\"ConnectorPlacement.EquallySpacedRectSide\",\"uuid\":\"1fb23197-7de0-4afe-988c-73e75d3e5644\"},{\"content\":{\"connectorIds\":[\"In1\"],\"side\":\"BOTTOM\"},\"type\":\"ConnectorPlacement.EquallySpacedRectSide\",\"uuid\":\"6caead23-812f-47a0-8d53-a65eccf1d005\"}]},\"type\":\"ConnectorPlacement.EquallySpacedConnector\",\"uuid\":\"0ef4e16f-7381-4a8b-98d2-b00a0700ad12\"}],\"packageUris\":[\"http://schema.mathworks.com/mf0/Connector/R2020b\"],\"version\":\"1.0\"}"
  Lane_select_App : Subsystem
      settings: PortSchema="{\"entries\":[{\"content\":{\"headerSize\":26,\"margin\":15,\"minimumSpacing\":25,\"sides\":[{\"content\":{\"connectorIds\":[\"In1\"]},\"type\":\"ConnectorPlacement.EquallySpacedRectSide\",\"uuid\":\"47be2e05-6379-4865-963e-e2af5bd447f4\"},{\"content\":{\"side\":\"RIGHT\"},\"type\":\"ConnectorPlacement.EquallySpacedRectSide\",\"uuid\":\"eee9a279-489d-42b1-868c-6501adb5baa4\"},{\"content\":{\"connectorIds\":[\"Out1\"],\"side\":\"TOP\"},\"type\":\"ConnectorPlacement.EquallySpacedRectSide\",\"uuid\":\"1fb23197-7de0-4afe-988c-73e75d3e5644\"}]},\"type\":\"ConnectorPlacement.EquallySpacedConnector\",\"uuid\":\"0ef4e16f-7381-4a8b-98d2-b00a0700ad12\"}],\"packageUris\":[\"http://schema.mathworks.com/mf0/Connector/R2020b\"],\"version\":\"1.0\"}"
  Parallel_Parking_App : Subsystem
      settings: PortSchema="{\"entries\":[{\"content\":{\"headerSize\":26,\"margin\":15,\"minimumSpacing\":25,\"sides\":[{\"content\":{\"connectorIds\":[\"In2\",\"In3\",\"In5\",\"In6\",\"In4\",\"In1\",\"In7\",\"In8\"]},\"type\":\"ConnectorPlacement.EquallySpacedRectSide\",\"uuid\":\"47be2e05-6379-4865-963e-e2af5bd447f4\"},{\"content\":{\"connectorIds\":[\"Out1\"],\"side\":\"RIGHT\"},\"type\":\"ConnectorPlacement.EquallySpacedRectSide\",\"uuid\":\"eee9a279-489d-42b1-868c-6501adb5baa4\"},{\"content\":{\"side\":\"TOP\"},\"type\":\"ConnectorPlacement.EquallySpacedRectSide\",\"uuid\":\"1fb23197-7de0-4afe-988c-73e75d3e5644\"}]},\"type\":\"ConnectorPlacement.EquallySpacedConnector\",\"uuid\":\"0ef4e16f-7381-4a8b-98d2-b00a0700ad12\"}],\"packageUris\":[\"http://schema.mathworks.com/mf0/Connector/R2020b\"],\"version\":\"1.0\"}"
  Sudden_Stop_App : Subsystem
      settings: PortSchema="{\"entries\":[{\"content\":{\"headerSize\":26,\"margin\":15,\"minimumSpacing\":25,\"sides\":[{\"content\":{\"connectorIds\":[\"In1\",\"In2\"]},\"type\":\"ConnectorPlacement.EquallySpacedRectSide\",\"uuid\":\"47be2e05-6379-4865-963e-e2af5bd447f4\"},{\"content\":{\"connectorIds\":[\"Out1\"],\"side\":\"RIGHT\"},\"type\":\"ConnectorPlacement.EquallySpacedRectSide\",\"uuid\":\"eee9a279-489d-42b1-868c-6501adb5baa4\"},{\"content\":{\"side\":\"TOP\"},\"type\":\"ConnectorPlacement.EquallySpacedRectSide\",\"uuid\":\"1fb23197-7de0-4afe-988c-73e75d3e5644\"}]},\"type\":\"ConnectorPlacement.EquallySpacedConnector\",\"uuid\":\"0ef4e16f-7381-4a8b-98d2-b00a0700ad12\"}],\"packageUris\":[\"http://schema.mathworks.com/mf0/Connector/R2020b\"],\"version\":\"1.0\"}"
  T_Parking_App : Subsystem
      settings: PortSchema="{\"entries\":[{\"content\":{\"headerSize\":26,\"margin\":15,\"minimumSpacing\":25,\"sides\":[{\"content\":{\"connectorIds\":[\"In1\",\"In2\",\"In4\",\"In5\",\"In3\",\"In6\",\"In7\",\"In8\"]},\"type\":\"ConnectorPlacement.EquallySpacedRectSide\",\"uuid\":\"47be2e05-6379-4865-963e-e2af5bd447f4\"},{\"content\":{\"connectorIds\":[\"Out1\"],\"side\":\"RIGHT\"},\"type\":\"ConnectorPlacement.EquallySpacedRectSide\",\"uuid\":\"eee9a279-489d-42b1-868c-6501adb5baa4\"},{\"content\":{\"side\":\"TOP\"},\"type\":\"ConnectorPlacement.EquallySpacedRectSide\",\"uuid\":\"1fb23197-7de0-4afe-988c-73e75d3e5644\"},{\"content\":{\"side\":\"BOTTOM\"},\"type\":\"ConnectorPlacement.EquallySpacedRectSide\",\"uuid\":\"97643e48-9f69-4ff0-bdfb-c04bf5b8c253\"}]},\"type\":\"ConnectorPlacement.EquallySpacedConnector\",\"uuid\":\"0ef4e16f-7381-4a8b-98d2-b00a0700ad12\"}],\"packageUris\":[\"http://schema.mathworks.com/mf0/Connector/R2020b\"],\"version\":\"1.0\"}"
  Traffic_App : Subsystem
      settings: PortSchema="{\"entries\":[{\"content\":{\"headerSize\":26,\"margin\":15,\"minimumSpacing\":25,\"sides\":[{\"content\":{\"connectorIds\":[\"In1\",\"In2\",\"In3\"]},\"type\":\"ConnectorPlacement.EquallySpacedRectSide\",\"uuid\":\"47be2e05-6379-4865-963e-e2af5bd447f4\"},{\"content\":{\"connectorIds\":[\"Out1\"],\"side\":\"RIGHT\"},\"type\":\"ConnectorPlacement.EquallySpacedRectSide\",\"uuid\":\"eee9a279-489d-42b1-868c-6501adb5baa4\"},{\"content\":{\"side\":\"TOP\"},\"type\":\"ConnectorPlacement.EquallySpacedRectSide\",\"uuid\":\"1fb23197-7de0-4afe-988c-73e75d3e5644\"}]},\"type\":\"ConnectorPlacement.EquallySpacedConnector\",\"uuid\":\"0ef4e16f-7381-4a8b-98d2-b00a0700ad12\"}],\"packageUris\":[\"http://schema.mathworks.com/mf0/Connector/R2020b\"],\"version\":\"1.0\"}"
  Bus Element Out1 : Outport  PortName=GPS_Trajectory
  Bus Element Out4 : Outport  Port=2  PortName=TParking_Trajectory
  Bus Element Out5 : Outport  Port=3  PortName=ParallelParking_Trajectory
  Bus Element Out3 : Outport  Port=4  PortName=Avoidance_Trajectory
  Bus Element Out2 : Outport  Port=5  PortName=Camera_Trajectory
  Bus Element Out6 : Outport  Port=6  PortName=MRM_Stop_Request
  Bus Element Out7 : Outport  Port=7  PortName=Traffic_Stop_Request
  wires:
  Bus Element In3/1 -> GPS_Driving_App/2(feedback_speed)
  Bus Element In6/1 -> Collision_Avoidance_App/1(feedback_speed)
  Bus Element In11/1 -> T_Parking_App/1(feedback_speed)
  Bus Element In8/1 -> Collision_Avoidance_App/2(feedback_steering_angle_deg)
  Bus Element In12/1 -> T_Parking_App/2(feedback_steering_angle_deg)
  Bus Element In7/1 -> GPS_Driving_App/6(feedback_steering_angle_deg)
  Bus Element In15/1 -> Parallel_Parking_App/2(feedback_speed)
  Bus Element In16/1 -> Parallel_Parking_App/3(feedback_steering_angle_deg)
  Bus Element In18/1 -> Camera_Driving_App/1(feedback_steering_angle_deg)
  Bus Element In19/1 -> Camera_Driving_App/2(feedback_speed)
  Bus Element In21/1 -> Sudden_Stop_App/1(feedback_speed)
  Bus Element In22/1 -> Traffic_App/3(feedback_speed)
  Lane_select_App/1(Lane_num) -> GPS_Driving_App/1(Lane_num)
  Collision_Avoidance_App/1(Avoidance_Trajectory) -> Bus Element Out3/1
  T_Parking_App/1(TParking_Trajectory) -> Bus Element Out4/1
  Parallel_Parking_App/1(ParallelParking_Trajectory) -> Bus Element Out5/1
  Sudden_Stop_App/1(MRM_Stop_Request) -> Bus Element Out6/1
  Traffic_App/1(Traffic_Stop_Request) -> Bus Element Out7/1
  GPS_Driving_App/1(Waypoint_Trajectory) -> Bus Element Out1/1
  Camera_Driving_App/1(Camera_Trajectory) -> Bus Element Out2/1
  Bus Element In5/1 -> Traffic_App/1("신호등 상태, 신호등 신뢰도")
  Bus Element In9/1 -> Traffic_App/2("정지선 검출 여부, 정지선 거리")
  Bus Element In10/1 -> Lane_select_App/1("신호차 상태, 신호차 신뢰도")
  Bus Element In13/1 -> GPS_Driving_App/3("현재 위치, 위치 정확도")
  Bus Element In14/1 -> GPS_Driving_App/4(GPS Fix 상태)
  Bus Element In17/1 -> GPS_Driving_App/5(RTK 상태)
  Bus Element In20/1 -> T_Parking_App/3("전방 연석 검출 여부, 측면 연석 거리")
  Bus Element In27/1 -> Parallel_Parking_App/4("전방 연석 검출 여부, 측면 연석 거리")
  Bus Element In23/1 -> T_Parking_App/4("주차공간 시작점, 끝점")
  Bus Element In28/1 -> Parallel_Parking_App/5("주차공간 시작점, 끝점")
  Bus Element In24/1 -> T_Parking_App/5(주차공간 길이)
  Bus Element In29/1 -> Parallel_Parking_App/6(주차공간 길이)
  Bus Element In25/1 -> Collision_Avoidance_App/3("전방 장애물 거리, 폭, 좌우 위치")
  Bus Element In31/1 -> Collision_Avoidance_App/4(주행 경로 내 장애물 여부)
  Bus Element In33/1 -> Sudden_Stop_App/2(주행 경로 내 장애물 여부)
  Bus Element In34/1 -> T_Parking_App/6(후방 연석 거리)
  Bus Element In35/1 -> T_Parking_App/7(후방 최종 정지 거리)
  Bus Element In36/1 -> Parallel_Parking_App/1(후방 안전거리)
  Bus Element In37/1 -> Parallel_Parking_App/7(후방 최종 정지 거리)
  Bus Element In38/1 -> Parallel_Parking_App/8(후방 연석 거리)
  Bus Element In39/1 -> Collision_Avoidance_App/5(후방 안전거리)
  Bus Element In40/1 -> T_Parking_App/8(후방 안전거리)
  Bus Element In4/1 -> Camera_Driving_App/4("3차 경로 계수, 경로 유효거리")
  Bus Element In2/1 -> Camera_Driving_App/3("차선/경로 유효 여부, 신뢰도, 차량 횡방향 오차")
  Bus Element In1/1 -> Camera_Driving_App/5("경로 방향 오차, 경로 곡률")

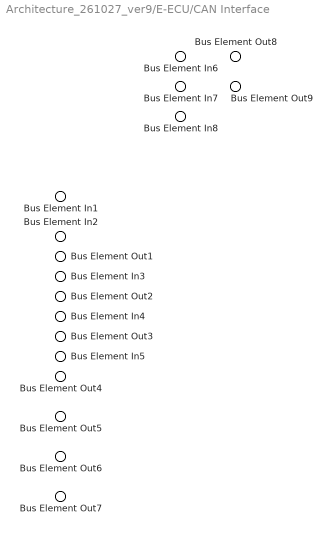
== system Architecture_261027_ver9/E-ECU/CAN Interface ==
  Bus Element In6 : Inport  PortName=Monitoring CAN
  Bus Element In1 : Inport  Port=2  PortName=Validated_GPS_Trajectory
  Bus Element In2 : Inport  Port=3  PortName=Validated_Camera_Trajectory
  Bus Element In3 : Inport  Port=4  PortName=Validated_TParking_Trajectory
  Bus Element In4 : Inport  Port=5  PortName=Validated_ParallelParking_Trajectory
  Bus Element In7 : Inport  Port=6  PortName=Validated_Traffic_Stop_Trajectory
  Bus Element In8 : Inport  Port=7  PortName=Validated_MRM_Stop_Trajectory
  Bus Element In5 : Inport  Port=8  PortName=Validated_Avoidance_Trajectory
  Bus Element Out8 : Outport  PortName=feedback_speed
  Bus Element Out9 : Outport  Port=2  PortName=feedback_steering_angle_deg
  Bus Element Out1 : Outport  Port=3  PortName=GPS_CANFD
  Bus Element Out2 : Outport  Port=4  PortName=Camera_CANFD
  Bus Element Out3 : Outport  Port=5  PortName=TParking_CANFD
  Bus Element Out4 : Outport  Port=6  PortName=ParallelParking_CANFD
  Bus Element Out5 : Outport  Port=7  PortName=Avoidance_CANFD
  Bus Element Out6 : Outport  Port=8  PortName=Traffic_Stop_CAN
  Bus Element Out7 : Outport  Port=9  PortName=MRM_Stop_CAN

== system Architecture_261027_ver9/E-ECU/CAN_FD ==
  Bus Element In7 : Inport  PortName=MRM_Stop_CAN
  Bus Element In6 : Inport  Port=2  PortName=Traffic_Stop_CAN
  Bus Element In1 : Inport  Port=3  PortName=GPS_CANFD
  Bus Element In2 : Inport  Port=4  PortName=Camera_CANFD
  Bus Element In3 : Inport  Port=5  PortName=TParking_CANFD
  Bus Element In4 : Inport  Port=6  PortName=ParallelParking_CANFD
  Bus Element In5 : Inport  Port=7  PortName=Avoidance_CANFD
  Bus Element Out1 : Outport  PortName=CANFD
